simulink model "matrix"  (R2025b)
settings: Solver=VariableStepAuto  StartTime=0.0  StopTime=10.0  RelTol=1e-3

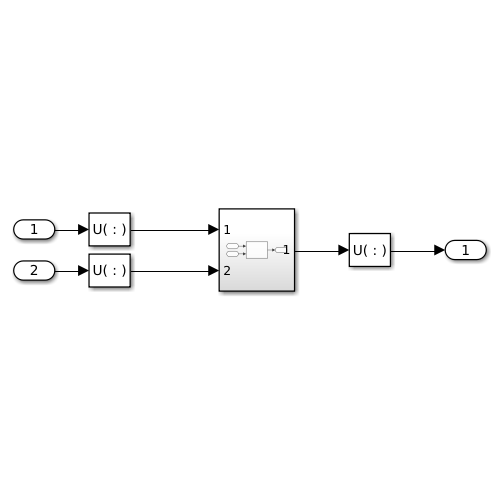
[thumbnail: Simulink's stored preview of the top-level diagram]
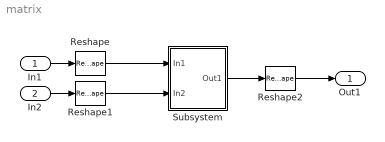
== system matrix ==
  In1 : Inport
  In2 : Inport  Port=2
  Reshape : Reshape
  Reshape1 : Reshape
  Reshape2 : Reshape
  Subsystem : Subsystem
  Out1 : Outport
  wires:
  Reshape/1 -> Subsystem/1(In1)
  In1/1 -> Reshape/1
  Reshape1/1 -> Subsystem/2(In2)
  In2/1 -> Reshape1/1
  Subsystem/1(Out1) -> Reshape2/1
  Reshape2/1 -> Out1/1

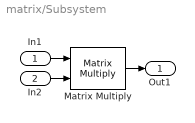
== system matrix/Subsystem ==
  In1 : Inport
  In2 : Inport  Port=2
  Matrix Multiply : Product  Multiplication=Matrix(*)
  Out1 : Outport
  wires:
  In1/1 -> Matrix Multiply/1
  In2/1 -> Matrix Multiply/2
  Matrix Multiply/1 -> Out1/1
